simulink model "x280_can_loopback"  (R2024b)
settings: Solver=FixedStepDiscrete  StartTime=0.0  StopTime=inf  FixedStep=0.001  RelTol=1e-3
InitFcn:
  | setupX280CANLibrary;
libraries: canmsglib x4
settings Model: Creator=Administrator  LastModifiedBy=Administrator
settings OptimizationCC: EnhancedBackFolding=on  PassReuseOutputArgsAs=Individual arguments  ZeroExternalMemoryAtStartup=off  ZeroInternalMemoryAtStartup=off  MaxStackSize=64  OptimizeBlockOrder=speed  DifferentSizesBufferReuse=on  OptimizationCustomize=off  EfficientTunableParamExpr=on
settings DebuggingCC: ParameterTunabilityLossMsg=error
settings HardwareCC: ProdBitPerLong=64  ProdHWDeviceType=Intel->x86-64 (Linux 64)
settings SFSimCC: MATLABDynamicMemAlloc=off
settings RTWCC: Description=Embedded Coder  SystemTargetFile=ert.tlc  HardwareBoard=SimRT  TLCOptions="-aInlineSetEventsForThisBaseRateFcn=TLC_FALSE -aSuppressMultiTaskScheduler=TLC_FALSE  -aRateBasedStepFcn=0"  TemplateMakefile=ert_default_tmf  Toolchain=X280 portable-linux-toolchain
settings CodeAppCC: ForceParamTrailComments=on  IgnoreCustomStorageClasses=off  OperatorAnnotations=on  SimulinkDataObjDesc=on  SFDataObjDesc=on  InsertBlockDesc=on
settings ERTTargetCC: ExtMode=on  ExtModeTransport=2  ExtModeStaticAlloc=on  ExtModeMexFile=ext_xcp  ExtModeIntrfLevel=Level2 - Open  InlinedParameterPlacement=Hierarchical

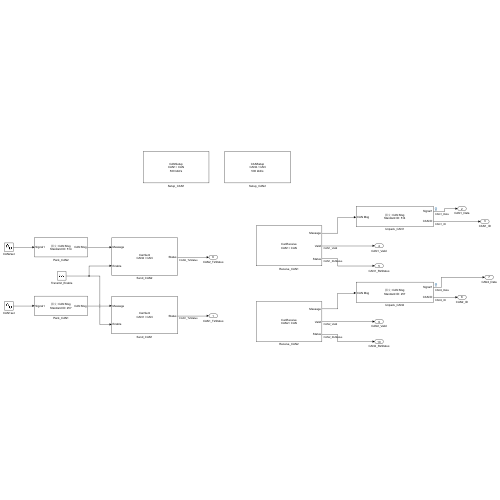
[thumbnail: Simulink's stored preview of the top-level diagram]
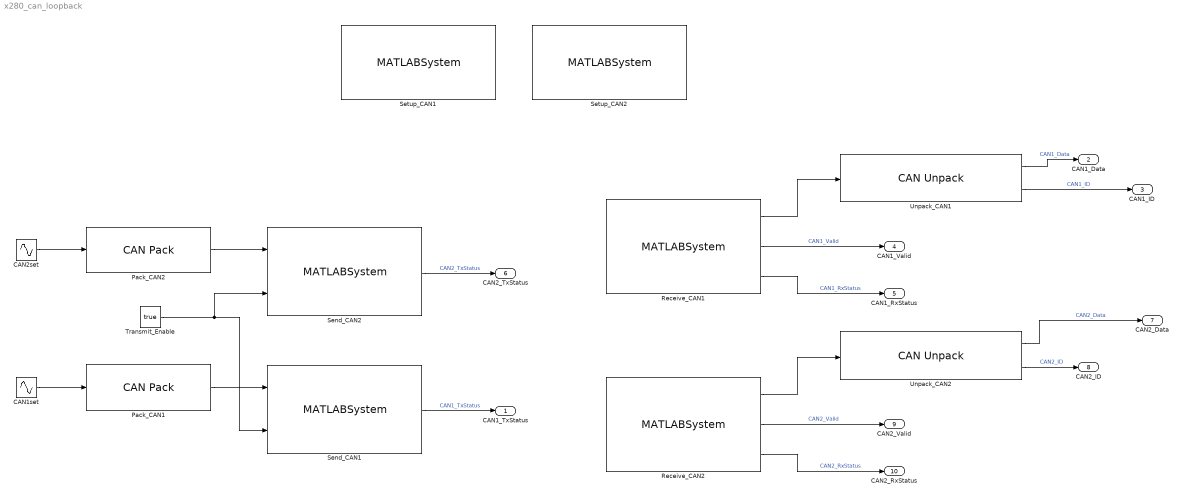
== system x280_can_loopback ==
  CAN1set : Sin  Amplitude=10  SampleTime=0.01
  CAN2set : Sin  Amplitude=10  SampleTime=0.01
  Pack_CAN1 : canmsglib/CAN Pack  MsgList=(none)  MsgName=CAN Msg  MsgIDType=Standard (11-bit identifier)  MsgIdentifier=257  CANIDInput=off  MsgLength=8  Remote=off  ApplyMinMax=off  BusOutput=on  SignalInfo={ 'Signal1', '0', '64', 'LE', 'double', 'Standard', '0', '1', '0', '-Inf', 'Inf' }
      settings: DataFormat=manually specified signals
  Pack_CAN2 : canmsglib/CAN Pack  MsgList=(none)  MsgName=CAN Msg  MsgIDType=Standard (11-bit identifier)  MsgIdentifier=514  CANIDInput=off  MsgLength=8  Remote=off  ApplyMinMax=off  BusOutput=on  SignalInfo={ 'Signal1', '0', '64', 'LE', 'double', 'Standard', '0', '1', '0', '-Inf', 'Inf' }
      settings: DataFormat=manually specified signals
  Receive_CAN1 : MATLABSystem  Priority=0  System=x280linux.can.CanReceive  Channel=1  CANType=CAN  SampleTime=0.001
      mask Type: x280linux.can.CanReceive
      mask Display:
      | disp(['CanReceive' char(10) 'CAN1 / CAN']);
      | port_label('output',1,'Message');
      | port_label('output',2,'Valid');
      | port_label('output',3,'Status');
  Receive_CAN2 : MATLABSystem  Priority=1  System=x280linux.can.CanReceive  Channel=2  CANType=CAN  SampleTime=0.001
      mask Type: x280linux.can.CanReceive
      mask Display:
      | disp(['CanReceive' char(10) 'CAN2 / CAN']);
      | port_label('output',1,'Message');
      | port_label('output',2,'Valid');
      | port_label('output',3,'Status');
  Send_CAN1 : MATLABSystem  Priority=-50  System=x280linux.can.CanSent  Channel=1  CANType=CAN
      mask Type: x280linux.can.CanSent
      mask Display:
      | disp(['CanSent' char(10) 'CAN1 / CAN']);
      | port_label('input',1,'Message');
      | port_label('input',2,'Enable');
      | port_label('output',1,'Status');
  Send_CAN2 : MATLABSystem  Priority=-49  System=x280linux.can.CanSent  Channel=2  CANType=CAN
      mask Type: x280linux.can.CanSent
      mask Display:
      | disp(['CanSent' char(10) 'CAN2 / CAN']);
      | port_label('input',1,'Message');
      | port_label('input',2,'Enable');
      | port_label('output',1,'Status');
  Setup_CAN1 : MATLABSystem  Priority=-100  System=x280linux.can.CANSetup  Channel=1  CANType=CAN  BaudRate=500  DataBitRate=2000  Termination=true  DriverDirectory=/home/zh/.local/lib/tscan-thread-fix-20260926  SampleTime=0.001  HostTransport=Loopback
      mask Type: x280linux.can.CANSetup
      mask Display: disp(['CANSetup' char(10) 'CAN1 / CAN' char(10) '500 kbit/s']);
  Setup_CAN2 : MATLABSystem  Priority=-99  System=x280linux.can.CANSetup  Channel=2  CANType=CAN  BaudRate=500  DataBitRate=2000  Termination=true  DriverDirectory=/home/zh/.local/lib/tscan-thread-fix-20260926  SampleTime=0.001  HostTransport=Loopback
      mask Type: x280linux.can.CANSetup
      mask Display: disp(['CANSetup' char(10) 'CAN2 / CAN' char(10) '500 kbit/s']);
  Transmit_Enable : Constant  Value=true  OutDataTypeStr=boolean  SampleTime=0.001
  Unpack_CAN1 : canmsglib/CAN Unpack  MsgList=(none)  MsgName=CAN Msg  MsgIDType=Standard (11-bit identifier)  MsgIdentifier=514  MsgLength=8  SignalInfo={ 'Signal1', '0', '64', 'LE', 'double', 'Standard', '0', '1', '0', '-Inf', 'Inf' }  IDPort=on  TimestampPort=off  ErrorPort=off  RemotePort=off  LengthPort=off  StatusPort=off  ApplyMinMax=off
  Unpack_CAN2 : canmsglib/CAN Unpack  MsgList=(none)  MsgName=CAN Msg  MsgIDType=Standard (11-bit identifier)  MsgIdentifier=257  MsgLength=8  SignalInfo={ 'Signal1', '0', '64', 'LE', 'double', 'Standard', '0', '1', '0', '-Inf', 'Inf' }  IDPort=on  TimestampPort=off  ErrorPort=off  RemotePort=off  LengthPort=off  StatusPort=off  ApplyMinMax=off
  CAN1_TxStatus : Outport
  CAN1_Data : Outport  Port=2
  CAN1_ID : Outport  Port=3
  CAN1_Valid : Outport  Port=4
  CAN1_RxStatus : Outport  Port=5
  CAN2_TxStatus : Outport  Port=6
  CAN2_Data : Outport  Port=7
  CAN2_ID : Outport  Port=8
  CAN2_Valid : Outport  Port=9
  CAN2_RxStatus : Outport  Port=10
  wires:
  Transmit_Enable/1 -> Send_CAN1/2, Send_CAN2/2
  Receive_CAN2/3 -> CAN2_RxStatus/1  "CAN2_RxStatus"
  Receive_CAN2/2 -> CAN2_Valid/1  "CAN2_Valid"
  Unpack_CAN2/2 -> CAN2_ID/1  "CAN2_ID"
  Unpack_CAN2/1 -> CAN2_Data/1  "CAN2_Data"
  Send_CAN2/1 -> CAN2_TxStatus/1  "CAN2_TxStatus"
  Receive_CAN2/1 -> Unpack_CAN2/1
  Pack_CAN2/1 -> Send_CAN2/1
  CAN2set/1 -> Pack_CAN2/1
  Receive_CAN1/3 -> CAN1_RxStatus/1  "CAN1_RxStatus"
  Receive_CAN1/2 -> CAN1_Valid/1  "CAN1_Valid"
  Unpack_CAN1/2 -> CAN1_ID/1  "CAN1_ID"
  Unpack_CAN1/1 -> CAN1_Data/1  "CAN1_Data"
  Send_CAN1/1 -> CAN1_TxStatus/1  "CAN1_TxStatus"
  Receive_CAN1/1 -> Unpack_CAN1/1
  Pack_CAN1/1 -> Send_CAN1/1
  CAN1set/1 -> Pack_CAN1/1
